simulink model "gfm_battery"  (R2018b)
settings: Solver=ode45  StartTime=0.0  StopTime=100  RelTol=1e-3
PreLoadFcn:
  | warning('STARTFCN ENTERED')
  | 
  | modelDir = fileparts(get_param(bdroot,'FileName'));
  | 
  | load_system(fullfile(modelDir,'controls_element_lib.slx'));
  | load_system(fullfile(modelDir,'test_sequence_lib.slx'));
  | 
  | warning('STARTFCN EXITED')
InitFcn:
  | close all;
  | clear all;
  | clc;
  | 
  | % frequency nominals
  | F_NOM = 60;
  | W_NOM = 2 * pi * F_NOM;
  | 
  | % base values relative to inverter
  | % --------------------------------
  | VLL_INV_NOM = 480;
  | P_INV_NOM = 1e6;
  | Q_INV_NOM = 0.5e6;
  | S_INV_NOM = sqrt(P_INV_NOM^2 + Q_INV_NOM^2);
  | 
  | I_INV_BASE = S_INV_NOM/(sqrt(3)*VLL_INV_NOM);
  | Z_INV_BASE = VLL_INV_NOM^2/S_INV_NOM;
  | L_INV_BASE = Z_INV_BASE / W_NOM;
  | C_INV_BASE = 1 / (Z_INV_BASE * W_NOM);
  | 
  | % nominal ratings for power system model
  | % --------------------------------------
  | INVERTER_COUNT = 100;
  | 
  | VLV_NOM = VLL_INV_NOM;
  | VMV_NOM = 35e3;
  | VHV_NOM = 230e3;
  | S_PLANT = INVERTER_COUNT * S_INV_NOM;
  | 
  | N_GSU = VHV_NOM/VMV_NOM;
  | N_MVT = VMV_NOM/VLV_NOM;
  | 
  | I_LV_BASE = S_PLANT/(sqrt(3)*VLV_NOM);
  | I_MV_BASE = S_PLANT/(sqrt(3)*VMV_NOM);
  | I_HV_BASE = S_PLANT/(sqrt(3)*VHV_NOM);
  | 
  | Z_LV_BASE = VLV_NOM^2/S_PLANT;
  | Z_MV_BASE = VMV_NOM^2/S_PLANT;
  | Z_HV_BASE = VHV_NOM^2/S_PLANT;
  | 
  | L_LV_BASE = Z_LV_BASE / W_NOM;
  | L_MV_BASE = Z_MV_BASE / W_NOM;
  | L_HV_BASE = Z_HV_BASE / W_NOM;
  | C_LV_BASE = 1 / (Z_LV_BASE * W_NOM);
  | C_MV_BASE = 1 / (Z_MV_BASE * W_NOM);
  | C_HV_BASE = 1 / (Z_HV_BASE * W_NOM);
libraries: test_sequence_lib x11, controls_element_lib x9
settings Model: SimulationMode=accelerator  Creator=halatrash  LastModifiedBy=ahhei
settings SolverCC: ZeroCrossAlgorithm=Adaptive
settings DataIOCC: ReturnWorkspaceOutputs=on
settings DebuggingCC: MaxConsecutiveZCsMsg=warning  IgnoredZcDiagnostic=none  UnconnectedInputMsg=none  UnconnectedOutputMsg=none  UnconnectedLineMsg=none
settings ModelReferenceCC: EnableRefExpFcnMdlSchedulingChecks=off
settings RTWCC: Description=Generic Real-Time Target
settings ConfigComp: CovBoundaryAbsTol=1.0e-5

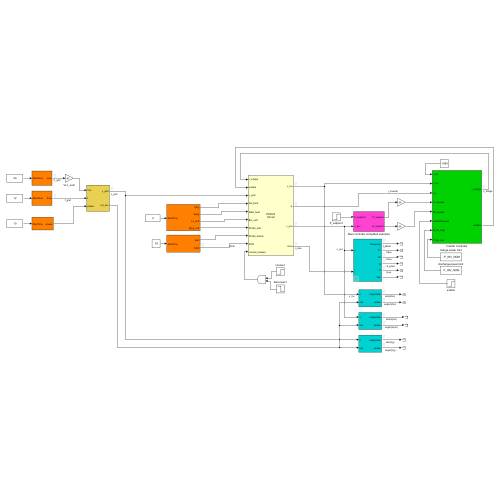
[thumbnail: Simulink's stored preview of the top-level diagram]
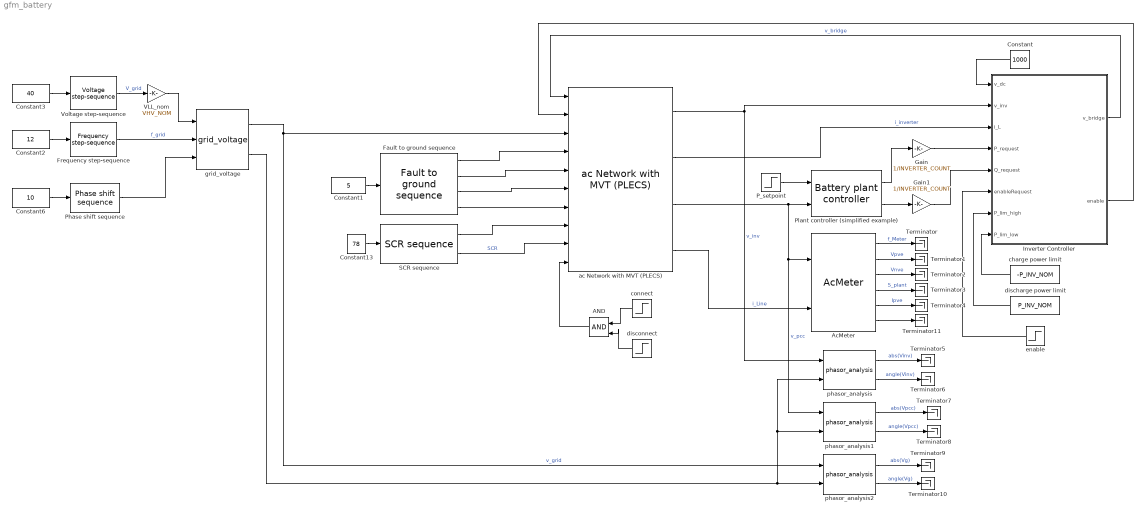
== system gfm_battery ==
  AND : Logic  IconShape=distinctive  AllPortsSameDT=off  OutDataTypeStr=boolean
  AcMeter : test_sequence_lib/AcMeter  VllRated=VHV_NOM
  Constant : Constant  Value=1000
  Constant1 : Constant  Value=5
  Constant13 : Constant  Value=78
  Constant2 : Constant  Value=12
  Constant3 : Constant  Value=40
  Constant6 : Constant  Value=10
  Fault to ground sequence : test_sequence_lib/Fault to ground sequence  SystemSampleTime=-1  EmptyChoice=off  PassThrough=off  PassThroughVariantControl=(default)  EmptyChoiceVariantControl=(default)  Latency=0  AutoFrameSizeCalculation=off
  Frequency step-sequence : test_sequence_lib/Frequency step-sequence  SystemSampleTime=-1  EmptyChoice=off  PassThrough=off  PassThroughVariantControl=(default)  EmptyChoiceVariantControl=(default)  Latency=0  AutoFrameSizeCalculation=off
  Gain : Gain  Gain=1/INVERTER_COUNT
  Gain1 : Gain  Gain=1/INVERTER_COUNT
  Inverter Controller : Subsystem
  P_setpoint : Step  Time=4  After=S_PLANT*0.5  SampleTime=0
  Phase shift sequence : test_sequence_lib/Phase shift sequence  SystemSampleTime=-1  EmptyChoice=off  PassThrough=off  PassThroughVariantControl=(default)  EmptyChoiceVariantControl=(default)  Latency=0  AutoFrameSizeCalculation=off
  Plant controller (simplified example) : controls_element_lib/Battery plant controller  SystemSampleTime=-1  EmptyChoice=off  PassThrough=off  PassThroughVariantControl=(default)  EmptyChoiceVariantControl=(default)  Latency=0  AutoFrameSizeCalculation=off
  SCR sequence : test_sequence_lib/SCR sequence  SystemSampleTime=-1  EmptyChoice=off  PassThrough=off  PassThroughVariantControl=(default)  EmptyChoiceVariantControl=(default)  Latency=0  AutoFrameSizeCalculation=off
  Terminator{,1..11} (12 alike) : Terminator
  VLL_nom : Gain  Gain=VHV_NOM
  Voltage step-sequence : test_sequence_lib/Voltage step-sequence  SystemSampleTime=-1  EmptyChoice=off  PassThrough=off  PassThroughVariantControl=(default)  EmptyChoiceVariantControl=(default)  Latency=0  AutoFrameSizeCalculation=off
  ac Network with MVT (PLECS) : test_sequence_lib/ac Network with MVT (PLECS)  PLECSData=<binary blob, 8620 chars, not shown>
  charge power limit : Constant  Value=-P_INV_NOM
  connect : Step  Time=0  SampleTime=0
  discharge power limit : Constant  Value=P_INV_NOM
  disconnect : Step  Time=97  Before=1  After=0  SampleTime=0
  enable : Step  Time=0.5  SampleTime=0
  grid_voltage : test_sequence_lib/grid_voltage  SystemSampleTime=-1  EmptyChoice=off  PassThrough=off  PassThroughVariantControl=(default)  EmptyChoiceVariantControl=(default)  Latency=0  AutoFrameSizeCalculation=off
  phasor_analysis : test_sequence_lib/phasor_analysis  SystemSampleTime=-1  EmptyChoice=off  PassThrough=off  PassThroughVariantControl=(default)  EmptyChoiceVariantControl=(default)  Latency=0  AutoFrameSizeCalculation=off
  phasor_analysis1 : test_sequence_lib/phasor_analysis  SystemSampleTime=-1  EmptyChoice=off  PassThrough=off  PassThroughVariantControl=(default)  EmptyChoiceVariantControl=(default)  Latency=0  AutoFrameSizeCalculation=off
  phasor_analysis2 : test_sequence_lib/phasor_analysis  SystemSampleTime=-1  EmptyChoice=off  PassThrough=off  PassThroughVariantControl=(default)  EmptyChoiceVariantControl=(default)  Latency=0  AutoFrameSizeCalculation=off
  wires:
  Constant13/1 -> SCR sequence/1
  AND/1 -> ac Network with MVT (PLECS)/10
  Constant3/1 -> Voltage step-sequence/1
  Constant2/1 -> Frequency step-sequence/1
  Phase shift sequence/1 -> grid_voltage/3
  Constant6/1 -> Phase shift sequence/1
  VLL_nom/1 -> grid_voltage/1
  Constant1/1 -> Fault to ground sequence/1
  Frequency step-sequence/1 -> grid_voltage/2  "f_grid"
  Voltage step-sequence/1 -> VLL_nom/1  "V_grid"
  SCR sequence/2 -> ac Network with MVT (PLECS)/9  "SCR"
  phasor_analysis1/1 -> Terminator7/1  "abs(Vpcc)"
  phasor_analysis1/2 -> Terminator8/1  "angle(Vpcc)"
  phasor_analysis/2 -> Terminator6/1  "angle(Vinv)"
  phasor_analysis2/2 -> Terminator10/1  "angle(Vg)"
  phasor_analysis/1 -> Terminator5/1  "abs(Vinv)"
  phasor_analysis2/1 -> Terminator9/1  "abs(Vg)"
  grid_voltage/2 -> phasor_analysis1/2, phasor_analysis/2, phasor_analysis2/2
  ac Network with MVT (PLECS)/1 -> Inverter Controller/2(v_inv), phasor_analysis/1  "v_inv"
  grid_voltage/1 -> ac Network with MVT (PLECS)/3, phasor_analysis2/1  "v_grid"
  Plant controller (simplified example)/2 -> Gain1/1
  ac Network with MVT (PLECS)/3 -> Plant controller (simplified example)/2, phasor_analysis1/1, AcMeter/1  "v_pcc"
  enable/1 -> Inverter Controller/6(enableRequest)
  connect/1 -> AND/1
  disconnect/1 -> AND/2
  ac Network with MVT (PLECS)/2 -> Inverter Controller/3(i_L)  "i_inverter"
  Plant controller (simplified example)/1 -> Gain/1
  P_setpoint/1 -> Plant controller (simplified example)/1
  AcMeter/1 -> Terminator/1  "f_Meter"
  AcMeter/5 -> Terminator4/1  "Ipve"
  AcMeter/3 -> Terminator2/1  "Vnve"
  AcMeter/2 -> Terminator1/1  "Vpve"
  AcMeter/4 -> Terminator3/1  "S_plant"
  Constant/1 -> Inverter Controller/1(v_dc)
  discharge power limit/1 -> Inverter Controller/7(P_lim_high)
  charge power limit/1 -> Inverter Controller/8(P_lim_low)
  AcMeter/6 -> Terminator11/1
  Inverter Controller/1(v_bridge) -> ac Network with MVT (PLECS)/1  "v_bridge"
  Inverter Controller/2(enable) -> ac Network with MVT (PLECS)/2
  Gain/1 -> Inverter Controller/4(P_request)
  Gain1/1 -> Inverter Controller/5(Q_request)
  SCR sequence/1 -> ac Network with MVT (PLECS)/8
  Fault to ground sequence/1 -> ac Network with MVT (PLECS)/4
  Fault to ground sequence/2 -> ac Network with MVT (PLECS)/5
  Fault to ground sequence/3 -> ac Network with MVT (PLECS)/6
  Fault to ground sequence/4 -> ac Network with MVT (PLECS)/7
  ac Network with MVT (PLECS)/4 -> AcMeter/2  "i_Line"

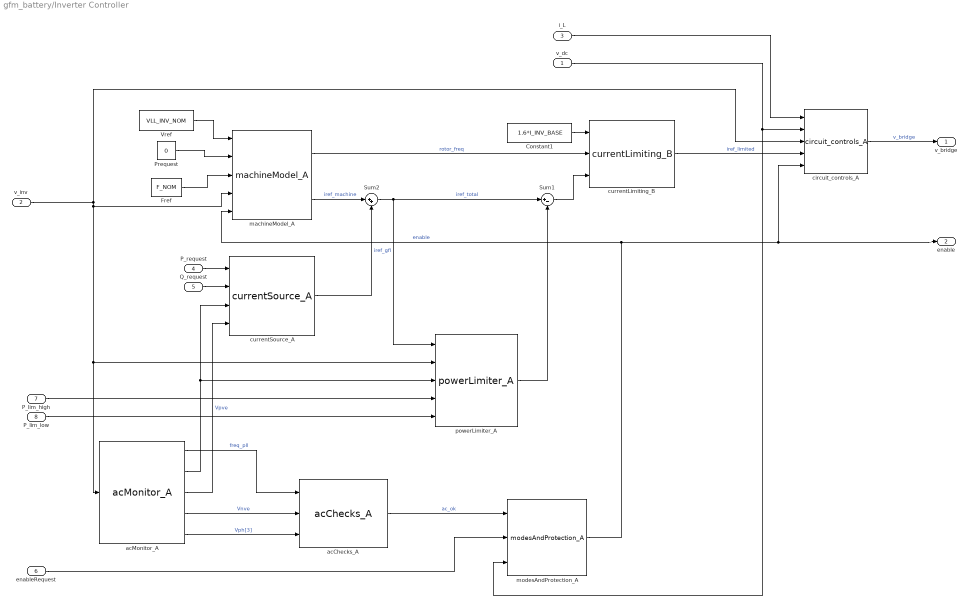
== system gfm_battery/Inverter Controller ==
  v_dc : Inport
  v_inv : Inport  Port=2
  i_L : Inport  Port=3
  P_request : Inport  Port=4
  Q_request : Inport  Port=5
  enableRequest : Inport  Port=6
  P_lim_high : Inport  Port=7
  P_lim_low : Inport  Port=8
  Constant1 : Constant  Value=1.6*I_INV_BASE
  Fref : Constant  Value=F_NOM
  Prequest : Constant  Value=0
  Sum1 : Sum  Inputs=|+-
  Sum2 : Sum  Inputs=|++
  Vref : Constant  Value=VLL_INV_NOM
  acChecks_A : controls_element_lib/acChecks_A  VllRated=VLL_INV_NOM  nominalFrequency=F_NOM  tRequalify=2  T_CNTL=1e-3
  "acMonitor_A " : controls_element_lib/acMonitor_A  VllRated=VLL_INV_NOM  nominalFrequency=F_NOM
  circuit_controls_A : controls_element_lib/circuit_controls_A  SystemSampleTime=-1  EmptyChoice=off  PassThrough=off  PassThroughVariantControl=(default)  EmptyChoiceVariantControl=(default)  Latency=0  AutoFrameSizeCalculation=off
  currentLimiting_B : controls_element_lib/currentLimiting_B  IRated=I_INV_BASE  peakSoftLimit=2.6  peakHardLimit=3.6
  currentSource_A : controls_element_lib/currentSource_A  VllRated=VLL_INV_NOM  SRated=S_INV_NOM  nominalFrequency=F_NOM  Plimit=P_INV_NOM/S_INV_NOM  Qlimit=Q_INV_NOM/S_INV_NOM
  machineModel_A : controls_element_lib/machineModel_A  SRated=S_INV_NOM  VllRated=VLL_INV_NOM  nominalFrequency=F_NOM  inertialConstant=2.5  kDroop=1  kDamper=2  Xs=0.3  rs=0.08  Qlimit=0.5  wExciter=10
  modesAndProtection_A : controls_element_lib/modesAndProtection_A  dcOvervotlageThreshold=1800  dcUndervotlageThreshold=700  dcTripClearTimeout=0.2
  powerLimiter_A : controls_element_lib/powerLimiter_A  VllRated=VLL_INV_NOM  nominalFrequency=F_NOM  wPowerLimiter=3
  v_bridge : Outport
  enable : Outport  Port=2
  wires:
  Vref/1 -> machineModel_A/1
  Prequest/1 -> machineModel_A/2
  Fref/1 -> machineModel_A/3
  machineModel_A/2 -> Sum2/1  "iref_machine"
  "acMonitor_A "/2 -> currentSource_A/3, powerLimiter_A/3
  currentLimiting_B/1 -> circuit_controls_A/4  "iref_limited"
  currentSource_A/1 -> Sum2/2  "iref_gfl"
  Sum2/1 -> Sum1/1, powerLimiter_A/1  "iref_total"
  "acMonitor_A "/3 -> currentSource_A/4  "Vpve"
  Q_request/1 -> currentSource_A/2
  P_request/1 -> currentSource_A/1
  enableRequest/1 -> modesAndProtection_A/2
  modesAndProtection_A/1 -> circuit_controls_A/5, enable/1, machineModel_A/5  "enable"
  "acMonitor_A "/5 -> acChecks_A/3  "Vph[3]"
  acChecks_A/1 -> modesAndProtection_A/1  "ac_ok"
  Constant1/1 -> currentLimiting_B/1
  "acMonitor_A "/1 -> acChecks_A/1  "freq_pll"
  "acMonitor_A "/4 -> acChecks_A/2  "Vnve"
  P_lim_low/1 -> powerLimiter_A/5
  P_lim_high/1 -> powerLimiter_A/4
  powerLimiter_A/1 -> Sum1/2
  Sum1/1 -> currentLimiting_B/3
  v_dc/1 -> circuit_controls_A/2, modesAndProtection_A/3
  circuit_controls_A/1 -> v_bridge/1  "v_bridge"
  machineModel_A/1 -> currentLimiting_B/2  "rotor_freq"
  i_L/1 -> circuit_controls_A/1
  v_inv/1 -> "acMonitor_A "/1, powerLimiter_A/2, machineModel_A/4, circuit_controls_A/3
